simulink model "DCDC_DAB_Converter"  (R2024b)
settings: Solver=ode23t  StartTime=0.0  StopTime=0.2  RelTol=1e-3
values from neighbouring files (symbols this model uses):
  C = I_out_DC / (votlage_ripple*fs)    (= 1.5625e-05)    [DAB_DCDC_Converter_Input_Parameter_Data.m]
  dt = Ts/100    (= 1e-07)    [DAB_DCDC_Converter_Input_Parameter_Data.m]
  fs = 100e3    (= 100000)    [DAB_DCDC_Converter_Input_Parameter_Data.m]
  L_act = L_req*FOS    (= 2.13333333333e-05)    [DAB_DCDC_Converter_Input_Parameter_Data.m]
  Pout = 30e3    (= 30000)    [DAB_DCDC_Converter_Input_Parameter_Data.m]
  R_load = Vout^2 / Pout    (= 21.3333333333)    [DAB_DCDC_Converter_Input_Parameter_Data.m]
  ratio_constant = selected_phi_time/Ts    [DAB_DCDC_Converter_Input_Parameter_Data.m]
  Vin = 800    [DAB_DCDC_Converter_Input_Parameter_Data.m]
  Vout = 800    [DAB_DCDC_Converter_Input_Parameter_Data.m]
libraries: spsMosfetLib x8, spsCurrentMeasurementLib x4, spsSeriesRLCBranchLib x3, spsVoltageMeasurementLib x3, spsMeanLib x2, slpidlib x2, spsDCVoltageSourceLib x1, spsGroundLib x1, spsLinearTransformerLib x1, spsRMSLib x1, sps_lib x1
settings Model: Creator=SUDHAK1  LastModifiedBy=SUDHAK1

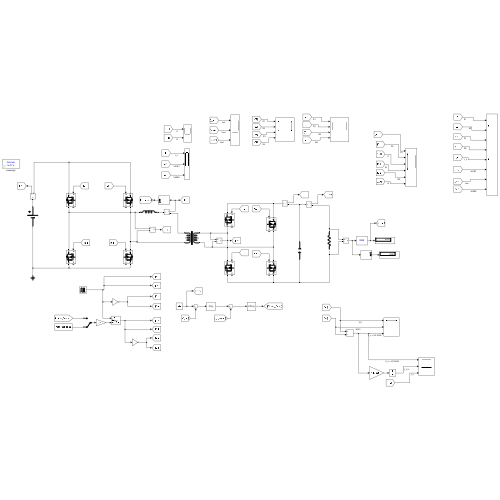
[thumbnail: Simulink's stored preview of the top-level diagram]
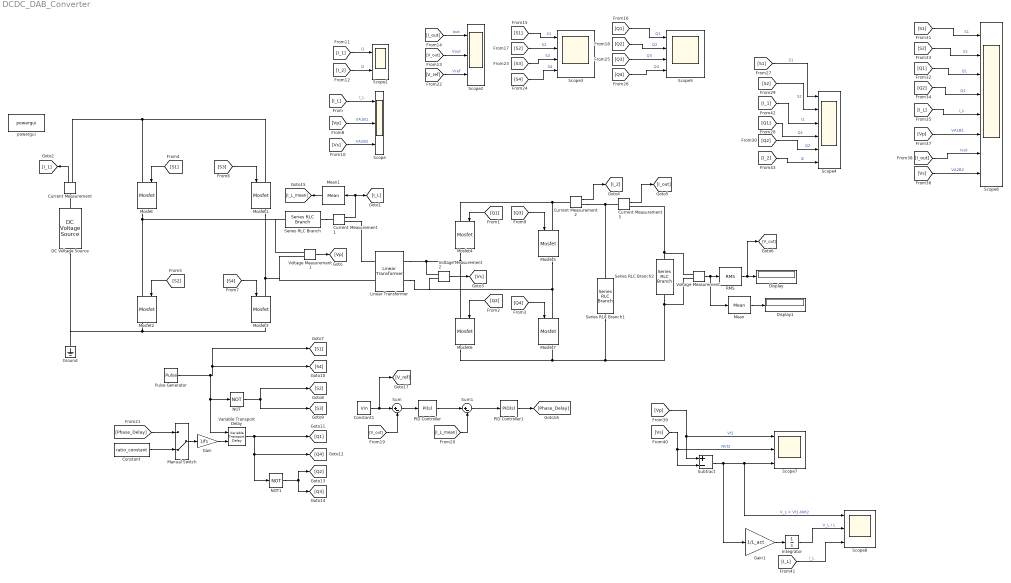
== system DCDC_DAB_Converter ==
  Constant : Constant  Value=ratio_constant
  Constant1 : Constant  Value=Vin
  Current Measurement{,1..3} (4 alike) : spsCurrentMeasurementLib/Current Measurement  PhasorSimulation=off  OutputType=Complex  PSBequivalent=0
  DC Voltage Source : spsDCVoltageSourceLib/DC Voltage Source  Amplitude=Vin  Measurements=None
  Display : Display
  Display1 : Display
  Gain : Gain  Gain=1/fs
  Gain1 : Gain  Gain=1/L_act
  Ground : spsGroundLib/Ground  LConnTagsString=a
  Integrator : Integrator
  Linear Transformer : spsLinearTransformerLib/Linear Transformer  UNITS=SI  NominalPower=[Pout fs]  winding1=[Vin 0 0]  winding2=[Vout 0 0]  ThreeWindings=off  winding3=[3.15e+05 0.7938 0.084225]  RmLm=[9.0038e+09 14330]  Measurements=None  DataType=on
  Manual Switch : ManualSwitch  CurrentSetting=0
  Mean : spsMeanLib/Mean  Freq=fs  Vinit=0  Ts=0
  Mean1 : spsMeanLib/Mean  Freq=60  Vinit=0  Ts=0
  Mosfet{,1..7} (8 alike) : spsMosfetLib/Mosfet  Ron=0.1  Lon=0  Rd=0.01  Vfd=0  IC=0  Rs=1e5  Cs=inf  Measurements=on
  NOT : Logic  Operator=NOT  IconShape=distinctive  AllPortsSameDT=off  OutDataTypeStr=boolean
  NOT1 : Logic  Operator=NOT  IconShape=distinctive  AllPortsSameDT=off  OutDataTypeStr=boolean
  PID Controller : slpidlib/PID Controller  Controller=PI  Form=Parallel  TimeDomain=Continuous-time  UseExternalTs=off  SampleTime=-1  IntegratorMethod=Forward Euler  FilterMethod=Forward Euler  ControllerParametersSource=internal  P=0.01  I=0.8  UseKiTs=off  D=0  UseExternalDerivativeSource=off  N=100  UseFilter=on  TunerSelectOption=Transfer Function Based (PID Tuner App)  InitialConditionSource=internal  InitialConditionForIntegrator=0  InitialConditionForFilter=0  DifferentiatorICPrevScaledInput=0  ExternalReset=none  TrackingMode=off  Kt=1  LimitOutput=off  SatLimitsSource=internal  UpperSaturationLimit=inf  LowerSaturationLimit=-inf  LinearizeAsGain=on  AntiWindupMode=none  Kb=1  LimitIntegrator=off  UpperIntegratorSaturationLimit=inf  LowerIntegratorSaturationLimit=-inf  POutMin=[]  POutMax=[]  IOutMin=[]  IOutMax=[]  DOutMin=[]  DOutMax=[]  NOutMin=[]  NOutMax=[]  SumOutMin=[]  SumOutMax=[]  SaturationOutMin=[]  SaturationOutMax=[]  PParamMin=[]  PParamMax=[]  IParamMin=[]  IParamMax=[]  DParamMin=[]  DParamMax=[]  NParamMin=[]  NParamMax=[]  KbParamMin=[]  KbParamMax=[]  KtParamMin=[]  KtParamMax=[]  KbOutMin=[]  KbOutMax=[]  KtOutMin=[]  KtOutMax=[]  IntegratorOutMin=[]  IntegratorOutMax=[]  FilterOutMin=[]  FilterOutMax=[]  SumI1OutMin=[]  SumI1OutMax=[]  SumI2OutMin=[]  SumI2OutMax=[]  SumI3OutMin=[]  SumI3OutMax=[]  SumI4OutMin=[]  SumI4OutMax=[]  SumDOutMin=[]  SumDOutMax=[]  DifferentiatorOutMin=[]  DifferentiatorOutMax=[]  FilterDiffOutCoefMin=[]  FilterDiffOutCoefMax=[]  ReciprocalOutMin=[]  ReciprocalOutMax=[]  SumDenOutMin=[]  SumDenOutMax=[]  SumNumOutMin=[]  SumNumOutMax=[]  DivideOutMin=[]  DivideOutMax=[]  UdiffTsProdOutMin=[]  UdiffTsProdOutMax=[]  NTsProdOutMin=[]  NTsProdOutMax=[]  UintegralTsProdOutMin=[]  UintegralTsProdOutMax=[]  UngainTsProdOutMin=[]  UngainTsProdOutMax=[]  ClampingZeroOutDataTypeStr=Inherit: Inherit via back propagation  ClampingZeroOutMin=[]  ClampingZeroOutMax=[]  FilterDenConstantOutDataTypeStr=Inherit: Inherit via back propagation  FilterDenConstantOutMin=[]  FilterDenConstantOutMax=[]  PCopyOutDataTypeStr=Inherit: Inherit via back propagation  PCopyOutMin=[]  PCopyOutMax=[]  NCopyOutDataTypeStr=Inherit: Inherit via back propagation  NCopyOutMin=[]  NCopyOutMax=[]  IntegratorContinuousStateAttributes=''  IntegratorStateMustResolveToSignalObject=off  IntegratorRTWStateStorageClass=Auto  FilterContinuousStateAttributes=''  FilterStateMustResolveToSignalObject=off  FilterRTWStateStorageClass=Auto  ParallelPVariant=InternalParameters  IdealPVariant=Disabled  IVariant=InternalParameters  DVariant=Disabled  IntegratorVariant=Continuous  SatVariant=Disabled  AWVariant=Passthrough  PCopyVariant=Disabled  TRVariant=Disabled  FdbkBlocksVariant=Forward  IdealPFdbkVariant=Disabled  SatFdbkVariant=Disabled  DerivativeFilterVariant=Disabled  NVariant=Disabled  NCopyVariant=Disabled_SignalSpec  FilterICVariant=Disabled  IntegratorICVariant=InternalICs  ExternalResetVariant=Disabled  TRSumVariant=Passthrough  SumFdbkVariant=Disabled  SumVariant=Sum_PI  TsampFilterVariant=InternalTs  TsampNgainVariant=Passthrough  TsampIntegralVariant=Disabled_SignalSpec  ExternalSaturationOutDataTypeStr=Inherit: Same as second input  DerivativeSourceVariant=Disabled  PreIntVariant=InternalPreInt
  PID Controller1 : slpidlib/PID Controller  Controller=PID  Form=Parallel  TimeDomain=Continuous-time  UseExternalTs=off  SampleTime=-1  IntegratorMethod=Forward Euler  FilterMethod=Forward Euler  ControllerParametersSource=internal  P=0.009  I=1  UseKiTs=off  D=0  UseExternalDerivativeSource=off  N=100  UseFilter=on  TunerSelectOption=Transfer Function Based (PID Tuner App)  InitialConditionSource=internal  InitialConditionForIntegrator=0  InitialConditionForFilter=0  DifferentiatorICPrevScaledInput=0  ExternalReset=none  TrackingMode=off  Kt=1  LimitOutput=off  SatLimitsSource=internal  UpperSaturationLimit=inf  LowerSaturationLimit=-inf  LinearizeAsGain=on  AntiWindupMode=none  Kb=1  LimitIntegrator=off  UpperIntegratorSaturationLimit=inf  LowerIntegratorSaturationLimit=-inf  POutMin=[]  POutMax=[]  IOutMin=[]  IOutMax=[]  DOutMin=[]  DOutMax=[]  NOutMin=[]  NOutMax=[]  SumOutMin=[]  SumOutMax=[]  SaturationOutMin=[]  SaturationOutMax=[]  PParamMin=[]  PParamMax=[]  IParamMin=[]  IParamMax=[]  DParamMin=[]  DParamMax=[]  NParamMin=[]  NParamMax=[]  KbParamMin=[]  KbParamMax=[]  KtParamMin=[]  KtParamMax=[]  KbOutMin=[]  KbOutMax=[]  KtOutMin=[]  KtOutMax=[]  IntegratorOutMin=[]  IntegratorOutMax=[]  FilterOutMin=[]  FilterOutMax=[]  SumI1OutMin=[]  SumI1OutMax=[]  SumI2OutMin=[]  SumI2OutMax=[]  SumI3OutMin=[]  SumI3OutMax=[]  SumI4OutMin=[]  SumI4OutMax=[]  SumDOutMin=[]  SumDOutMax=[]  DifferentiatorOutMin=[]  DifferentiatorOutMax=[]  FilterDiffOutCoefMin=[]  FilterDiffOutCoefMax=[]  ReciprocalOutMin=[]  ReciprocalOutMax=[]  SumDenOutMin=[]  SumDenOutMax=[]  SumNumOutMin=[]  SumNumOutMax=[]  DivideOutMin=[]  DivideOutMax=[]  UdiffTsProdOutMin=[]  UdiffTsProdOutMax=[]  NTsProdOutMin=[]  NTsProdOutMax=[]  UintegralTsProdOutMin=[]  UintegralTsProdOutMax=[]  UngainTsProdOutMin=[]  UngainTsProdOutMax=[]  ClampingZeroOutDataTypeStr=Inherit: Inherit via back propagation  ClampingZeroOutMin=[]  ClampingZeroOutMax=[]  FilterDenConstantOutDataTypeStr=Inherit: Inherit via back propagation  FilterDenConstantOutMin=[]  FilterDenConstantOutMax=[]  PCopyOutDataTypeStr=Inherit: Inherit via back propagation  PCopyOutMin=[]  PCopyOutMax=[]  NCopyOutDataTypeStr=Inherit: Inherit via back propagation  NCopyOutMin=[]  NCopyOutMax=[]  IntegratorContinuousStateAttributes=''  IntegratorStateMustResolveToSignalObject=off  IntegratorRTWStateStorageClass=Auto  FilterContinuousStateAttributes=''  FilterStateMustResolveToSignalObject=off  FilterRTWStateStorageClass=Auto  ParallelPVariant=InternalParameters  IdealPVariant=Disabled  IVariant=InternalParameters  DVariant=InternalParameters  IntegratorVariant=Continuous  SatVariant=Disabled  AWVariant=Passthrough  PCopyVariant=Disabled  TRVariant=Disabled  FdbkBlocksVariant=Forward  IdealPFdbkVariant=Disabled  SatFdbkVariant=Disabled  DerivativeFilterVariant=ContFilter  NVariant=InternalParameters  NCopyVariant=Disabled  FilterICVariant=InternalICsFilter  IntegratorICVariant=InternalICs  ExternalResetVariant=Disabled  TRSumVariant=Passthrough  SumFdbkVariant=Disabled  SumVariant=Sum_PID  TsampFilterVariant=InternalTs  TsampNgainVariant=Passthrough  TsampIntegralVariant=Disabled_SignalSpec  ExternalSaturationOutDataTypeStr=Inherit: Same as second input  DerivativeSourceVariant=ErrorSignal  PreIntVariant=InternalPreInt
  Pulse Generator : DiscretePulseGenerator  PulseType=Time based  Period=1/fs  PulseWidth=50
  RMS : spsRMSLib/RMS  TrueRMS=on  Freq=60  RMSInit=120  Ts=0
  Scope{,2,7..8} (4 alike) : Scope  NumInputPorts=3
  Scope1 : Scope  NumInputPorts=2
  Scope3 : Scope  NumInputPorts=4
  Scope4 : Scope  NumInputPorts=6
  Scope5 : Scope  NumInputPorts=4
  Scope6 : Scope  NumInputPorts=8
  Series RLC Branch : spsSeriesRLCBranchLib/Series RLC Branch  LConnTagsString=__new0  RConnTagsString=__new0  BranchType=L  Resistance=1  Inductance=L_act  SetiL0=off  InitialCurrent=0  Capacitance=1e-6  Setx0=off  InitialVoltage=0  Measurements=None
  Series RLC Branch1 : spsSeriesRLCBranchLib/Series RLC Branch  LConnTagsString=__new0  RConnTagsString=__new0  BranchType=C  Resistance=1  Inductance=7.8e-7  SetiL0=off  InitialCurrent=0  Capacitance=C*2  Setx0=off  InitialVoltage=0  Measurements=None
  Series RLC Branch2 : spsSeriesRLCBranchLib/Series RLC Branch  LConnTagsString=__new0  RConnTagsString=__new0  BranchType=R  Resistance=R_load  Inductance=1e-3  SetiL0=off  InitialCurrent=0  Capacitance=1e-6  Setx0=off  InitialVoltage=0  Measurements=None
  Subtract : Sum  Inputs=+-
  Sum : Sum  Inputs=|+-
  Sum1 : Sum  Inputs=|+-
  Variable Transport Delay : VariableTransportDelay  VariableDelayType=Variable transport delay  MaximumDelay=10
  Voltage Measurement : spsVoltageMeasurementLib/Voltage Measurement  PhasorSimulation=off  OutputType=Complex  PSBequivalent=0
  Voltage Measurement1 : spsVoltageMeasurementLib/Voltage Measurement  PhasorSimulation=off  OutputType=Complex  PSBequivalent=0
  Voltage Measurement2 : spsVoltageMeasurementLib/Voltage Measurement  PhasorSimulation=off  OutputType=Complex  PSBequivalent=0
  powergui : sps_lib/powergui  Priority=1  SimulationMode=Discrete  SampleTime=dt  frequency=60  Iterations=50  frequencyindice=0  Pbase=100e6  ErrMax=1e-4  UnitsV=kV  UnitsW=MW  buscounter=0  FunctionMessages=off  echomessages=off  EnableUseOfTLC=off  CurrentSourceSwitches=off  DisableSnubberDevices=off  DisableRonSwitches=off  DisableVfSwitches=off  DisplayEquations=off  AutomaticDiscreteSolvers=off  SolverType=Tustin/Backward Euler (TBE)  Interpol=off  ExternalGateDelay=off  methode=off  Ts=100  x0status=blocks  SPID=on  SwTol=0  HookPort=off  NonlinearTolerance=1e-4  nMaxIteration=100  ContinueOnMaxIteration=off  RestoreLinks=warning  ResistiveCurrentMeasurement=off  Frange=[0:2:500]  Ylog=off  Xlog=on  ShowGrid=off  save=off  variable=ZData  structure=0  ZoomFFT=off  StartTime=0.0  cycles=1  DisplayStyle=1  fundamental=60  FreqAxis=off  MaxFrequency=1000  frequencyindicesteady=1  RmsSteady=1  display=off
  wires:
  [S2] -> Mosfet2/1
  [S4] -> Mosfet3/1
  Voltage Measurement/1 -> RMS/1, Mean/1
  RMS/1 -> [V_out], Display/1
  [S1] -> Mosfet/1
  [S3] -> Mosfet1/1
  Voltage Measurement1/1 -> [Vp]
  Current Measurement1/1 -> Mean1/1, [I_L]
  Current Measurement/1 -> [I_1]
  Voltage Measurement2/1 -> [Vs]
  [I_L] -> Scope/1  "I_L"
  [Vp] -> Scope/2  "VA1B1"
  [Vs] -> Scope/3  "VA2B2"
  [I_1] -> Scope1/1  "I1"
  Current Measurement2/1 -> [I_2]
  [I_2] -> Scope1/2  "I2"
  [I_out] -> Scope2/1  "Iout"
  [V_out] -> Scope2/2  "Vout"
  Pulse Generator/1 -> Variable Transport Delay/1, NOT/1, [S1], [S4]
  NOT/1 -> [S2], [S3]
  NOT1/1 -> [Q3], [Q2]
  Variable Transport Delay/1 -> [Q1], [Q4], NOT1/1
  Current Measurement3/1 -> [I_out]
  Mean/1 -> Display1/1
  Constant1/1 -> [V_ref], Sum/1
  [V_out] -> Sum/2
  Sum/1 -> PID Controller/1
  PID Controller/1 -> Sum1/1
  Mean1/1 -> [I_L_mean]
  [I_L_mean] -> Sum1/2
  Sum1/1 -> PID Controller1/1
  PID Controller1/1 -> [Phase_Delay]
  Constant/1 -> Manual Switch/2
  [Phase_Delay] -> Manual Switch/1
  Manual Switch/1 -> Gain/1
  Gain/1 -> Variable Transport Delay/2
  [V_ref] -> Scope2/3  "Vref"
  [Q2] -> Mosfet6/1
  [Q4] -> Mosfet7/1
  [Q1] -> Mosfet4/1
  [Q3] -> Mosfet5/1
  [S1] -> Scope3/1  "S1"
  [S2] -> Scope3/2  "S2"
  [S3] -> Scope3/3  "S3"
  [S4] -> Scope3/4  "S4"
  [Q1] -> Scope5/1  "Q1"
  [Q2] -> Scope5/2  "Q2"
  [Q3] -> Scope5/3  "Q3"
  [Q4] -> Scope5/4  "Q4"
  [Q2] -> Scope4/5  "Q2"
  [S1] -> Scope4/1  "S1"
  [Q1] -> Scope4/4  "Q1"
  [S2] -> Scope4/2  "S2"
  [S1] -> Scope6/1  "S1"
  [Q2] -> Scope6/4  "Q2"
  [S2] -> Scope6/2  "S2"
  [Q1] -> Scope6/3  "Q1"
  [Vs] -> Scope6/8  "VA2B2"
  [I_L] -> Scope6/5  "I_L"
  [Vp] -> Scope6/6  "VA1B1"
  [I_out] -> Scope6/7  "Iout"
  [Vp] -> Scope7/1, Subtract/1  "Vt1"
  [Vs] -> Scope7/2, Subtract/2  "NVt2"
  Subtract/1 -> Gain1/1, Scope8/1, Scope7/3  "V_L = Vt1-NVt2"
  Gain1/1 -> Integrator/1
  Integrator/1 -> Scope8/2  "V_L / L"
  [I_L] -> Scope8/3  "I_L"
  [I_2] -> Scope4/6  "I2"
  [I_1] -> Scope4/3  "I1"
  connections:
  Mosfet/RConn1 -- Voltage Measurement1/LConn1 -- Series RLC Branch/LConn1 -- Mosfet2/LConn1
  Mosfet1/RConn1 -- Voltage Measurement1/LConn2 -- Linear Transformer/LConn2 -- Mosfet3/LConn1
  DC Voltage Source/RConn1 -- Current Measurement/LConn1
  Mosfet2/RConn1 -- Ground/LConn1 -- DC Voltage Source/LConn1 -- Mosfet3/RConn1
  Current Measurement/RConn1 -- Mosfet1/LConn1 -- Mosfet/LConn1
  Series RLC Branch/RConn1 -- Current Measurement1/LConn1
  Current Measurement1/RConn1 -- Linear Transformer/LConn1
  Current Measurement2/RConn1 -- Series RLC Branch1/LConn1 -- Current Measurement3/LConn1
  Voltage Measurement/LConn1 -- Current Measurement3/RConn1 -- Series RLC Branch2/LConn1
  Linear Transformer/RConn1 -- Voltage Measurement2/LConn1 -- Mosfet6/LConn1 -- Mosfet4/RConn1
  Mosfet4/LConn1 -- Current Measurement2/LConn1 -- Mosfet5/LConn1
  Series RLC Branch1/RConn1 -- Voltage Measurement/LConn2 -- Series RLC Branch2/RConn1 -- Mosfet6/RConn1 -- Mosfet7/RConn1
  Mosfet5/RConn1 -- Voltage Measurement2/LConn2 -- Linear Transformer/RConn2 -- Mosfet7/LConn1
